simulink model "aura_mission"  (R2026b)
settings: Solver=ode4  StopTime=stopTime  FixedStep=fixedStep
values from neighbouring files (symbols this model uses):
  Area = [2 2 3 3 6 6 3 3 3 3] * 1e-2    [main.m]
  e0 = [deg2rad(180) deg2rad(0) deg2rad(0)]'    [main.m]
  ecc = 0.001    [main.m]
  fixedStep = 0.1    [main.m]
  I = diag([Ix Iy Iz])    [main.m]
  I_inv = inv(I)    [main.m]
  inc = deg2rad(30)    [main.m]
  j_B = [0.01 0.05 0.01]    [main.m]
  mu_E = astroConstants(13)    [main.m]
  N_B = [ 1  0  0 ... (first row only)    [main.m]
  omega0 = [deg2rad(0) deg2rad(0) n]'    [main.m]
  r_F = r_geo - r_cm    [main.m]
  rho_d = [0 0 0 0 0.25 0.25 0.25 0.25 0 0]    [main.m]
  rho_s = [0 0 0 0 0.10 0.10 0.10 0.10 0 0]    [main.m]
  sma = R_E + height    [main.m]
  ta0 = 0    [main.m]
  usePerts = 1    [main.m]
undefined symbols (not defined in the file or in its folder): w_0
libraries: library x18, matrix_library x1
settings Model: Creator=bonoms  LastModifiedBy=bonoms

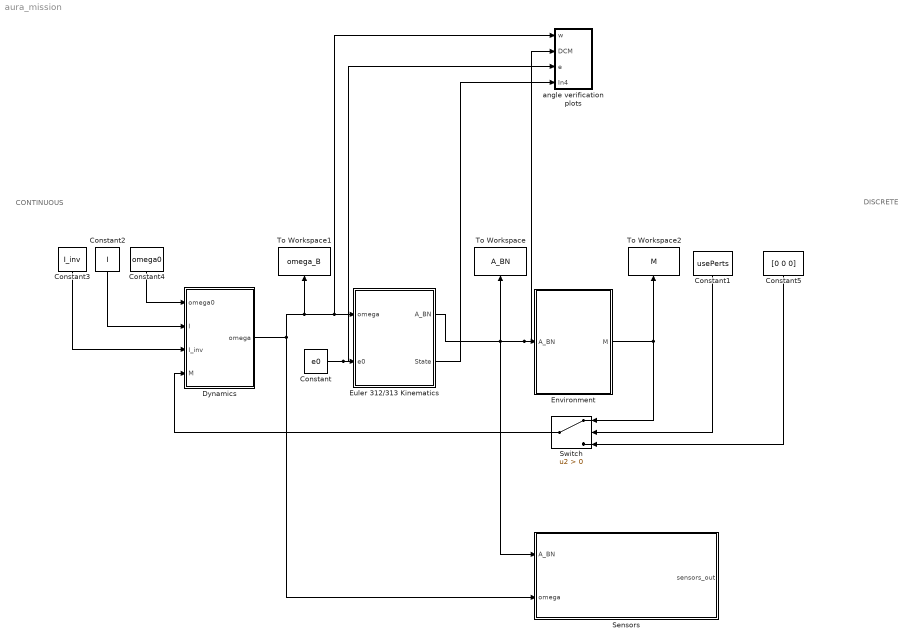
== system aura_mission ==
  note: DISCRETE
  note: CONTINUOUS
  Constant : Constant  Value=e0
  Constant1 : Constant  Value=usePerts
  Constant2 : Constant  Value=I
  Constant3 : Constant  Value=I_inv
  Constant4 : Constant  Value=omega0
  Constant5 : Constant  Value=[0 0 0]
  Dynamics : Subsystem
  Environment : Subsystem
  Euler 312/313 Kinematics : Subsystem
  Sensors : Subsystem
  Switch : Switch  Criteria=u2 > Threshold  SaturateOnIntegerOverflow=off  InputSameDT=off
  To Workspace : ToWorkspace  VariableName=A_BN  SampleTime=-1
  To Workspace1 : ToWorkspace  VariableName=omega_B  SampleTime=-1
  To Workspace2 : ToWorkspace  VariableName=M  SampleTime=-1
  angle verification plots : Subsystem
  wires:
  Dynamics/1(omega) -> Sensors/2(omega), Euler 312/313 Kinematics/1(omega), angle verification plots/1(w), To Workspace1/1
  Constant2/1 -> Dynamics/2(I)
  Constant4/1 -> Dynamics/1(omega0)
  Constant3/1 -> Dynamics/3(I_inv)
  Constant/1 -> angle verification plots/3(e), Euler 312/313 Kinematics/2(e0)
  Euler 312/313 Kinematics/1(A_BN) -> angle verification plots/2(DCM), Environment/1(A_BN), To Workspace/1, Sensors/1(A_BN)
  Environment/1(M) -> Switch/1, To Workspace2/1
  Constant1/1 -> Switch/2
  Switch/1 -> Dynamics/4(M)
  Constant5/1 -> Switch/3
  Euler 312/313 Kinematics/2(State) -> angle verification plots/4(In4)

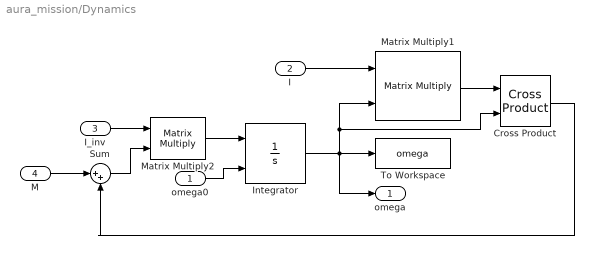
== system aura_mission/Dynamics ==
  omega0 : Inport
  I : Inport  Port=2
  I_inv : Inport  Port=3
  M : Inport  Port=4
  Cross Product : matrix_library/Cross Product
  Integrator : Integrator  InitialConditionSource=external  InitialCondition=w_0
  Matrix Multiply1 : Product  Multiplication=Matrix(*)
  Matrix Multiply2 : Product  Multiplication=Matrix(*)
  Sum : Sum  Inputs=|++
  To Workspace : ToWorkspace  VariableName=omega  SampleTime=-1
  omega : Outport
  wires:
  Matrix Multiply1/1 -> Cross Product/1
  Integrator/1 -> Matrix Multiply1/2, Cross Product/2, To Workspace/1, omega/1
  omega0/1 -> Integrator/2
  Sum/1 -> Matrix Multiply2/2
  I/1 -> Matrix Multiply1/1
  Matrix Multiply2/1 -> Integrator/1
  I_inv/1 -> Matrix Multiply2/1
  Cross Product/1 -> Sum/2
  M/1 -> Sum/1

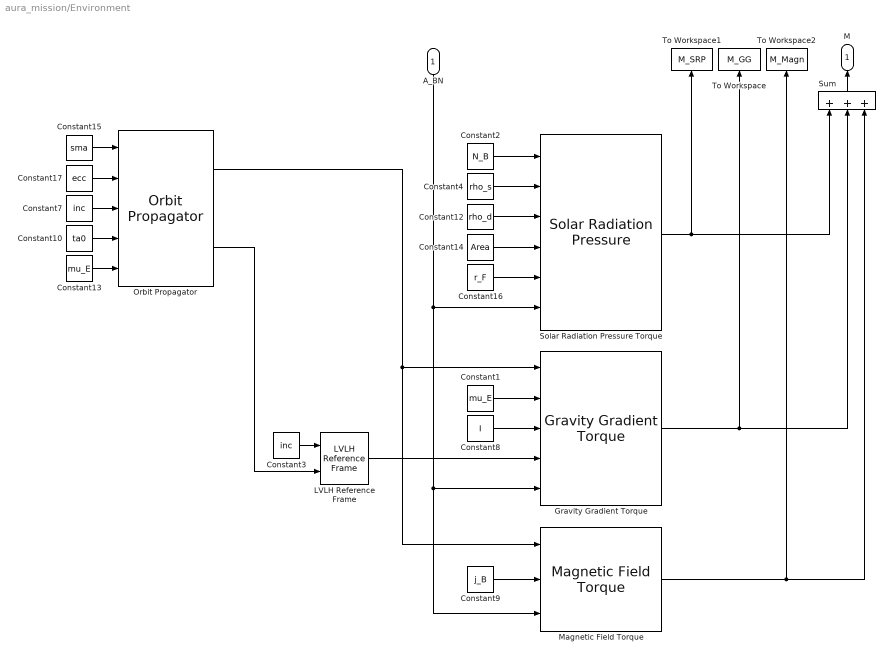
== system aura_mission/Environment ==
  A_BN : Inport
  Constant1 : Constant  Value=mu_E
  Constant10 : Constant  Value=ta0
  Constant12 : Constant  Value=rho_d
  Constant13 : Constant  Value=mu_E
  Constant14 : Constant  Value=Area
  Constant15 : Constant  Value=sma
  Constant16 : Constant  Value=r_F
  Constant17 : Constant  Value=ecc
  Constant2 : Constant  Value=N_B
  Constant3 : Constant  Value=inc
  Constant4 : Constant  Value=rho_s
  Constant7 : Constant  Value=inc
  Constant8 : Constant  Value=I
  Constant9 : Constant  Value=j_B
  Gravity Gradient Torque : library/Gravity Gradient Torque  SystemSampleTime=-1  VariantActivationTime=update diagram  EmptyChoice=off  PassThrough=off  PassThroughVariantControl=(default)  EmptyChoiceVariantControl=(default)  AllowFlexibleInterface=on  Latency=0  AutoFrameSizeCalculation=off
      settings: SourceProductName=SAD Project
  LVLH Reference Frame : library/LVLH Reference Frame  Description=Inputs: theta_rad (true anomaly), inclination_rad; scalar angles in radians. Output: 3x3 A_LN = Rz_passive(theta)*Rx_passive(i). Maps inertial columns to radial/transverse/normal axes for RAAN=argument of periapsis=0. Exactly the supplied matrix product. No workspace variables.  SystemSampleTime=-1  VariantActivationTime=update diagram  EmptyChoice=off  PassThrough=off  PassThroughVariantControl=(default)  EmptyChoiceVariantControl=(default)  AllowFlexibleInterface=on  Latency=0  AutoFrameSizeCalculation=off
      settings: SourceProductName=SAD Project
  Magnetic Field Torque : library/Magnetic Field Torque  SystemSampleTime=-1  VariantActivationTime=update diagram  EmptyChoice=off  PassThrough=off  PassThroughVariantControl=(default)  EmptyChoiceVariantControl=(default)  AllowFlexibleInterface=on  Latency=0  AutoFrameSizeCalculation=off
      link override Earth magnetic dipole tilt: Value=2.00712e-01
      settings: SourceProductName=SAD Project
  Orbit Propagator : library/Orbit Propagator  SystemSampleTime=-1  VariantActivationTime=update diagram  EmptyChoice=off  PassThrough=off  PassThroughVariantControl=(default)  EmptyChoiceVariantControl=(default)  AllowFlexibleInterface=on  Latency=0  AutoFrameSizeCalculation=off
      settings: SourceProductName=SAD Project
  Solar Radiation Pressure Torque : library/Solar Radiation Pressure  SystemSampleTime=-1  VariantActivationTime=update diagram  EmptyChoice=off  PassThrough=off  PassThroughVariantControl=(default)  EmptyChoiceVariantControl=(default)  AllowFlexibleInterface=on  Latency=0  AutoFrameSizeCalculation=off
      settings: SourceProductName=SAD Project
  Sum : Sum  Inputs=+++
  To Workspace : ToWorkspace  VariableName=M_GG  SampleTime=-1
  To Workspace1 : ToWorkspace  VariableName=M_SRP  SampleTime=-1
  To Workspace2 : ToWorkspace  VariableName=M_Magn  SampleTime=-1
  M : Outport
  wires:
  A_BN/1 -> Magnetic Field Torque/3, Gravity Gradient Torque/5, Solar Radiation Pressure Torque/6
  Constant2/1 -> Solar Radiation Pressure Torque/1
  Constant4/1 -> Solar Radiation Pressure Torque/2
  Constant12/1 -> Solar Radiation Pressure Torque/3
  Constant14/1 -> Solar Radiation Pressure Torque/4
  Constant16/1 -> Solar Radiation Pressure Torque/5
  Constant8/1 -> Gravity Gradient Torque/3
  Constant1/1 -> Gravity Gradient Torque/2
  Constant9/1 -> Magnetic Field Torque/2
  Constant15/1 -> Orbit Propagator/1
  Constant17/1 -> Orbit Propagator/2
  Constant10/1 -> Orbit Propagator/4
  Constant13/1 -> Orbit Propagator/5
  Orbit Propagator/1 -> Magnetic Field Torque/1, Gravity Gradient Torque/1
  LVLH Reference Frame/1 -> Gravity Gradient Torque/4
  Orbit Propagator/2 -> LVLH Reference Frame/2
  Constant7/1 -> Orbit Propagator/3
  Constant3/1 -> LVLH Reference Frame/1
  Solar Radiation Pressure Torque/1 -> Sum/1, To Workspace1/1
  Gravity Gradient Torque/1 -> Sum/2, To Workspace/1
  Magnetic Field Torque/1 -> Sum/3, To Workspace2/1
  Sum/1 -> M/1

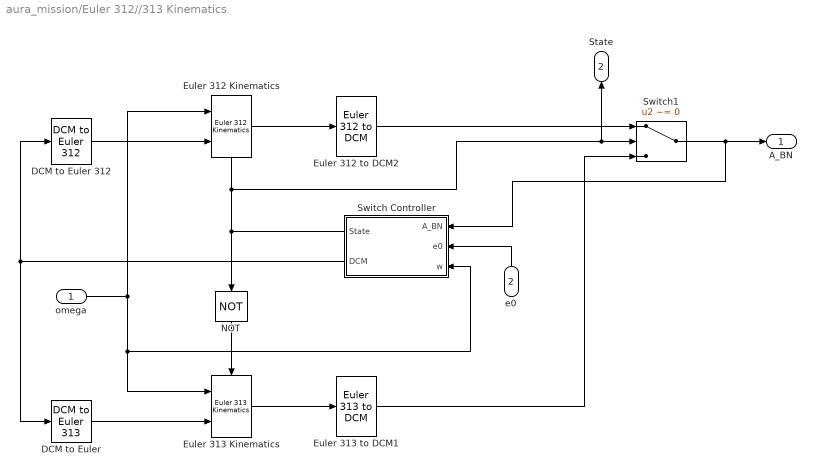
== system aura_mission/Euler 312//313 Kinematics ==
  omega : Inport
  e0 : Inport  Port=2
  DCM to Euler : library/DCM to Euler 313  SystemSampleTime=-1  VariantActivationTime=update diagram  EmptyChoice=off  PassThrough=off  PassThroughVariantControl=(default)  EmptyChoiceVariantControl=(default)  AllowFlexibleInterface=on  Latency=0  AutoFrameSizeCalculation=off
      settings: SourceProductName=SAD Project
  DCM to Euler 312 : library/DCM to Euler 312  SystemSampleTime=-1  VariantActivationTime=update diagram  EmptyChoice=off  PassThrough=off  PassThroughVariantControl=(default)  EmptyChoiceVariantControl=(default)  AllowFlexibleInterface=on  Latency=0  AutoFrameSizeCalculation=off
      settings: SourceProductName=SAD Project
  Euler 312 Kinematics : library/Euler 312 Kinematics  SystemSampleTime=-1  VariantActivationTime=update diagram  EmptyChoice=off  PassThrough=off  PassThroughVariantControl=(default)  EmptyChoiceVariantControl=(default)  AllowFlexibleInterface=on  Latency=0  AutoFrameSizeCalculation=off
      settings: SourceProductName=SAD Project
  Euler 312 to DCM2 : library/Euler 312 to DCM  SystemSampleTime=-1  VariantActivationTime=update diagram  EmptyChoice=off  PassThrough=off  PassThroughVariantControl=(default)  EmptyChoiceVariantControl=(default)  AllowFlexibleInterface=on  Latency=0  AutoFrameSizeCalculation=off
      settings: SourceProductName=SAD Project
  Euler 313 Kinematics : library/Euler 313 Kinematics  SystemSampleTime=-1  VariantActivationTime=update diagram  EmptyChoice=off  PassThrough=off  PassThroughVariantControl=(default)  EmptyChoiceVariantControl=(default)  AllowFlexibleInterface=on  Latency=0  AutoFrameSizeCalculation=off
      settings: SourceProductName=SAD Project
  Euler 313 to DCM1 : library/Euler 313 to DCM  SystemSampleTime=-1  VariantActivationTime=update diagram  EmptyChoice=off  PassThrough=off  PassThroughVariantControl=(default)  EmptyChoiceVariantControl=(default)  AllowFlexibleInterface=on  Latency=0  AutoFrameSizeCalculation=off
      settings: SourceProductName=SAD Project
  NOT : Logic  Operator=NOT  IconShape=distinctive  AllPortsSameDT=off  OutDataTypeStr=boolean
  Switch Controller : Subsystem
  Switch1 : Switch  Criteria=u2 ~= 0  SaturateOnIntegerOverflow=off  InputSameDT=off
  A_BN : Outport
  State : Outport  Port=2
  wires:
  DCM to Euler 312/1 -> Euler 312 Kinematics/2
  Switch1/1 -> A_BN/1, Switch Controller/1(A_BN)
  omega/1 -> Euler 312 Kinematics/1, Euler 313 Kinematics/1, Switch Controller/3(w)
  Euler 313 to DCM1/1 -> Switch1/3
  Switch Controller/1(State) -> Euler 312 Kinematics/Enable, State/1, Switch1/2, NOT/1
  Switch Controller/2(DCM) -> DCM to Euler 312/1, DCM to Euler/1
  e0/1 -> Switch Controller/2(e0)
  Euler 312 to DCM2/1 -> Switch1/1
  Euler 312 Kinematics/1 -> Euler 312 to DCM2/1
  Euler 313 Kinematics/1 -> Euler 313 to DCM1/1
  NOT/1 -> Euler 313 Kinematics/Enable
  DCM to Euler/1 -> Euler 313 Kinematics/2

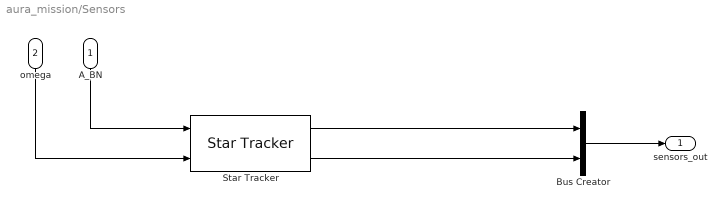
== system aura_mission/Sensors ==
  A_BN : Inport
  omega : Inport  Port=2
  Bus Creator : BusCreator  Inputs=2
  Star Tracker : library/Star Tracker  SystemSampleTime=-1  VariantActivationTime=update diagram  EmptyChoice=off  PassThrough=off  PassThroughVariantControl=(default)  EmptyChoiceVariantControl=(default)  AllowFlexibleInterface=on  Latency=0  AutoFrameSizeCalculation=off
      settings: SourceProductName=SAD Project
  sensors_out : Outport
  wires:
  A_BN/1 -> Star Tracker/1
  omega/1 -> Star Tracker/2
  Bus Creator/1 -> sensors_out/1
  Star Tracker/1 -> Bus Creator/1
  Star Tracker/2 -> Bus Creator/2

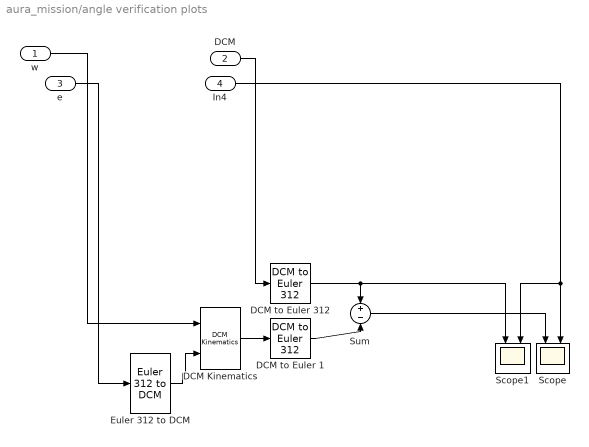
== system aura_mission/angle verification plots ==
  w : Inport
  DCM : Inport  Port=2
  e : Inport  Port=3
  In4 : Inport  Port=4
  DCM Kinematics : library/DCM Kinematics  SystemSampleTime=-1  VariantActivationTime=update diagram  EmptyChoice=off  PassThrough=off  PassThroughVariantControl=(default)  EmptyChoiceVariantControl=(default)  AllowFlexibleInterface=on  Latency=0  AutoFrameSizeCalculation=off
      settings: SourceProductName=SAD Project
  DCM to Euler 1 : library/DCM to Euler 312  SystemSampleTime=-1  VariantActivationTime=update diagram  EmptyChoice=off  PassThrough=off  PassThroughVariantControl=(default)  EmptyChoiceVariantControl=(default)  AllowFlexibleInterface=on  Latency=0  AutoFrameSizeCalculation=off
      settings: SourceProductName=SAD Project
  DCM to Euler 312 : library/DCM to Euler 312  SystemSampleTime=-1  VariantActivationTime=update diagram  EmptyChoice=off  PassThrough=off  PassThroughVariantControl=(default)  EmptyChoiceVariantControl=(default)  AllowFlexibleInterface=on  Latency=0  AutoFrameSizeCalculation=off
      settings: SourceProductName=SAD Project
  Euler 312 to DCM : library/Euler 312 to DCM  SystemSampleTime=-1  VariantActivationTime=update diagram  EmptyChoice=off  PassThrough=off  PassThroughVariantControl=(default)  EmptyChoiceVariantControl=(default)  AllowFlexibleInterface=on  Latency=0  AutoFrameSizeCalculation=off
      settings: SourceProductName=SAD Project
  Scope : Scope  NumInputPorts=2
      settings: ActiveDisplayYMinimum=-1.1089569013688392  ActiveDisplayYMaximum=2.3157149502021164
  Scope1 : Scope  NumInputPorts=2
      settings: ActiveDisplayYMinimum=-3.926984332287788  ActiveDisplayYMaximum=3.9269536557464382
  Sum : Sum  Inputs=+|-
  wires:
  e/1 -> Euler 312 to DCM/1
  w/1 -> DCM Kinematics/1
  DCM to Euler 1/1 -> Sum/2
  In4/1 -> Scope1/2, Scope/2
  DCM/1 -> DCM to Euler 312/1
  DCM Kinematics/1 -> DCM to Euler 1/1
  Sum/1 -> Scope/1
  Euler 312 to DCM/1 -> DCM Kinematics/2
  DCM to Euler 312/1 -> Scope1/1, Sum/1

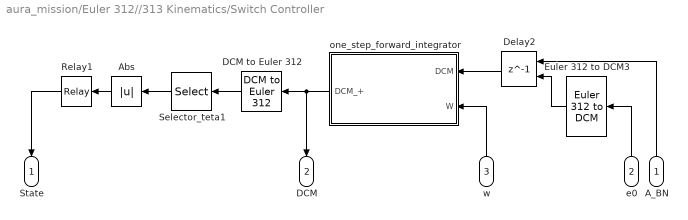
== system aura_mission/Euler 312//313 Kinematics/Switch Controller ==
  A_BN : Inport
  e0 : Inport  Port=2
  w : Inport  Port=3
  Abs : Abs  SaturateOnIntegerOverflow=off
  DCM to Euler 312 : library/DCM to Euler 312  SystemSampleTime=-1  VariantActivationTime=update diagram  EmptyChoice=off  PassThrough=off  PassThroughVariantControl=(default)  EmptyChoiceVariantControl=(default)  AllowFlexibleInterface=on  Latency=0  AutoFrameSizeCalculation=off
      settings: SourceProductName=SAD Project
  Delay2 : Delay  DelayLength=1  InitialConditionSource=Input port
      settings: InputPortMap=u0,p4
  Euler 312 to DCM3 : library/Euler 312 to DCM  SystemSampleTime=-1  VariantActivationTime=update diagram  EmptyChoice=off  PassThrough=off  PassThroughVariantControl=(default)  EmptyChoiceVariantControl=(default)  AllowFlexibleInterface=on  Latency=0  AutoFrameSizeCalculation=off
      settings: SourceProductName=SAD Project
  Relay1 : Relay  OnSwitchValue=deg2rad(60)  OffSwitchValue=deg2rad(30)  OnOutputValue=0  OffOutputValue=1
  Selector_teta1 : Selector  InputPortWidth=3  IndexOptions=Index vector (dialog)  Indices=2  OutputSizes=1  RuntimeRangeChecks=off
  one_step_forward_integrator : Subsystem
  State : Outport
  DCM : Outport  Port=2
  wires:
  w/1 -> one_step_forward_integrator/2(W)
  Delay2/1 -> one_step_forward_integrator/1(DCM)
  one_step_forward_integrator/1(DCM_+) -> DCM to Euler 312/1, DCM/1
  Relay1/1 -> State/1
  Abs/1 -> Relay1/1
  e0/1 -> Euler 312 to DCM3/1
  DCM to Euler 312/1 -> Selector_teta1/1
  Euler 312 to DCM3/1 -> Delay2/2
  A_BN/1 -> Delay2/1
  Selector_teta1/1 -> Abs/1

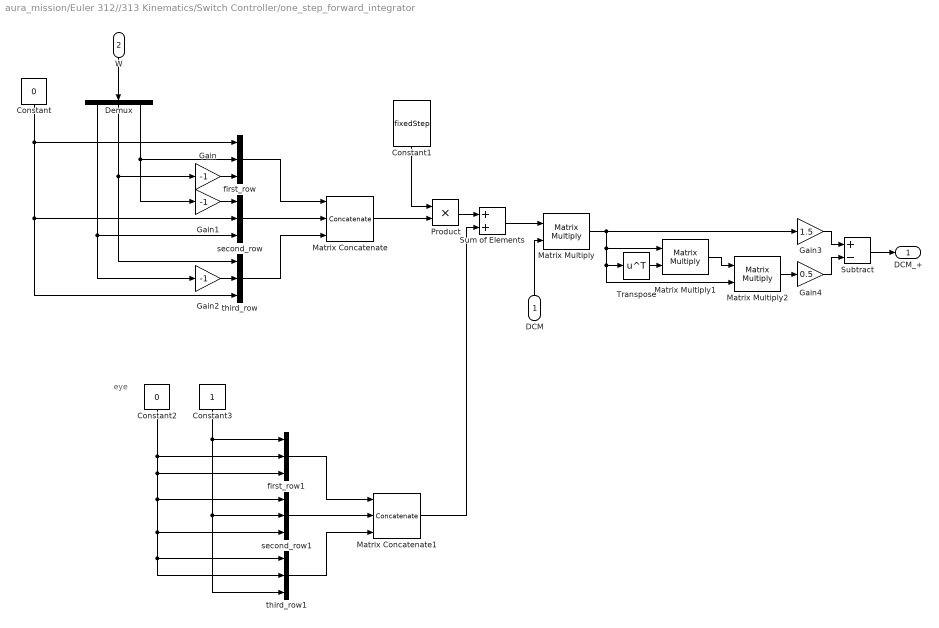
== system aura_mission/Euler 312//313 Kinematics/Switch Controller/one_step_forward_integrator ==
  note: eye
  DCM : Inport
  W : Inport  Port=2
  Constant : Constant  Value=0
  Constant1 : Constant  Value=fixedStep
  Constant2 : Constant  Value=0
  Constant3 : Constant
  Demux : Demux  Outputs=3
  Gain : Gain  Gain=-1
  Gain1 : Gain  Gain=-1
  Gain2 : Gain  Gain=-1
  Gain3 : Gain  Gain=1.5
  Gain4 : Gain  Gain=0.5
  Matrix Concatenate : Concatenate  NumInputs=3  Mode=Multidimensional array  ConcatenateDimension=2
  Matrix Concatenate1 : Concatenate  NumInputs=3  Mode=Multidimensional array  ConcatenateDimension=2
  Matrix Multiply : Product  Multiplication=Matrix(*)
  Matrix Multiply1 : Product  Multiplication=Matrix(*)
  Matrix Multiply2 : Product  Multiplication=Matrix(*)
  Product : Product
  Subtract : Sum  Inputs=+-
  Sum of Elements : Sum
  Transpose : Math  Operator=transpose
  first_row : Mux  Inputs=3
  first_row1 : Mux  Inputs=3
  second_row : Mux  Inputs=3
  second_row1 : Mux  Inputs=3
  third_row : Mux  Inputs=3
  third_row1 : Mux  Inputs=3
  DCM_+ : Outport
  wires:
  Gain2/1 -> third_row/2
  Matrix Concatenate1/1 -> Sum of Elements/2
  Constant2/1 -> second_row1/3, third_row1/1, third_row1/2, second_row1/1, first_row1/3, first_row1/2
  Constant3/1 -> second_row1/2, third_row1/3, first_row1/1
  third_row1/1 -> Matrix Concatenate1/3
  second_row1/1 -> Matrix Concatenate1/2
  first_row1/1 -> Matrix Concatenate1/1
  Sum of Elements/1 -> Matrix Multiply/1
  Product/1 -> Sum of Elements/1
  Matrix Concatenate/1 -> Product/2
  W/1 -> Demux/1
  Constant1/1 -> Product/1
  DCM/1 -> Matrix Multiply/2
  Demux/1 -> second_row/3, Gain2/1
  Gain1/1 -> second_row/1
  Demux/2 -> Gain/1, third_row/1
  Gain/1 -> first_row/3
  Demux/3 -> Gain1/1, first_row/2
  Constant/1 -> third_row/3, second_row/2, first_row/1
  first_row/1 -> Matrix Concatenate/1
  second_row/1 -> Matrix Concatenate/2
  third_row/1 -> Matrix Concatenate/3
  Gain4/1 -> Subtract/2
  Matrix Multiply1/1 -> Matrix Multiply2/1
  Matrix Multiply2/1 -> Gain4/1
  Transpose/1 -> Matrix Multiply1/2
  Gain3/1 -> Subtract/1
  Matrix Multiply/1 -> Matrix Multiply2/2, Transpose/1, Matrix Multiply1/1, Gain3/1
  Subtract/1 -> DCM_+/1
